simulink library "Linkage_DW_A"  (R2026a)
settings: Solver=VariableStepAuto
undefined symbols (not defined in the file): Ac, Af, Ar, InitLinkage, Left, Linkage, Visual, X, Y, Z
libraries: sm_lib x49, Suspension_Utilities x22, Linkage_Shock x1, fl_lib x1, nesl_utility x1
(part 1 of 2)
Description:
  | Component of Simscape Vehicle Templates Library
  | 
  | Copyright 2018-2024 The MathWorks, Inc.
settings Model: Creator=smiller  LastModifiedBy=andrei

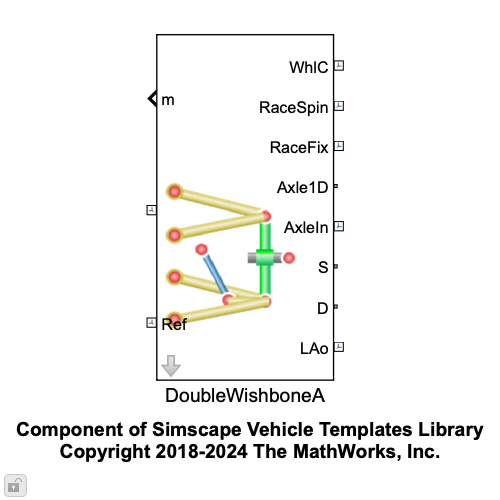
[thumbnail: Simulink's stored preview of the top-level diagram]
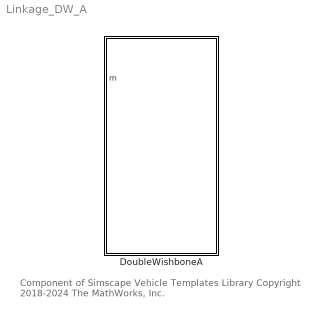
== system Linkage_DW_A ==
  note: Component of Simscape Vehicle Templates Library
      | Copyright 2018-2024 The MathWorks, Inc.
  DoubleWishboneA : Subsystem  VariantControl=DoubleWishboneA  mask(Double-Wishbone Suspension, Design A){popup_leftRight=Left, hp_in_f_ua=Linkage.UpperWishbone.sInboardF.Value, hp_in_r_ua=Linkage.UpperWishbone.sInboardR.Value, hp_out_ua=Linkage.UpperWishbone.sOutboard.Value, hp_in_f_la=Linkage.LowerWishbone.sInboardF.Value, hp_in_r_la=Linkage.LowerWishbone.sInboardR.Value, hp_out_la=Linkage.LowerWishbone.sOutboard.Value, hp_upr_cg=Linkage.Upright.sCG.Value, hp_upr_wc=Linkage.Upright.sWheelCentre.Value, hp_in_rod=Linkage.TrackRod.sInboard.Value, hp_upr_rod=Linkage.TrackRod.sOutboard.Value, hp_spr_top=Linkage.Shock.sTop.Value, hp_spr_bot=Linkage.Shock.sBottom.Value, clr_hp=Visual.hp.clr, opc_hp=Visual.hp.opc, size_hp=Visual.hp.rad, Upper_Arm_to_Subframe=Linkage.Upper_Arm_to_Subframe, ua_mass=Linkage.UpperWishbone.m.Value, clr_ua=Visual.UpperArm.clr, opc_ua=Visual.part.opc, radius_ua=Visual.UpperArm.rad, Lower_Arm_to_Subframe=Linkage.Lower_Arm_to_Subframe, la_mass=Linkage.LowerWishbone.m.Value, clr_la=Visual.LowerArm.clr, opc_la=Visual.part.opc, radius_la=Visual.LowerArm.rad, shock_pist_mass=Linkage.Shock.mPiston.Value, shock_cyl_mass=Linkage.Shock.mCylinder.Value, up_lim_bumpstop=Linkage.Endstop.xMax.Value, low_lim_bumpstop=Linkage.Endstop.xMin.Value, clr_conn_shock=Visual.hp.clr, opc_conn_shock=Visual.hp.opc, size_conn_shock=Visual.hp.rad, clr_shock_cyl=Visual.Shock.cyl.clr, opc_shock_cyl=Visual.part.opc, radius_shock_cyl=Visual.Shock.cyl.rad, clr_shock_piston=Visual.Shock.piston.clr, opc_shock_piston=Visual.part.opc, clr_shock_bumpstop=Visual.Shock.bumpstop.clr, opc_shock_bumpstop=Visual.part.opc, deadvol_len_shock_cyl=Visual.Shock.dead_length, piston_len_shock=Visual.Shock.piston.len, cyl_cap_len_shock=Visual.Shock.cap.len, bumpstop_len_shock=Visual.Shock.bumpstop.len, atoe=Linkage.Upright.aToe.Value, acamber=Linkage.Upright.aCamber.Value, upr_mass=Linkage.Upright.m.Value, axle_len=Linkage.Upright.xAxle.Value, axle_whlc_to_bearing=Linkage.Upright.xWCtoBearing.Value, axle_mass=Linkage.Upright.mAxle.Value, clr_conn_upr=Visual.hp.clr, opc_conn_upr=Visual.hp.opc, size_conn_upr=Visual.hp.rad, clr_upr=Visual.Upright.clr, opc_upr=Visual.part.opc, radius_upr=Visual.Upright.rad, clr_axle=Visual.Axle.clr, opc_axle=Visual.part.opc, radius_axle=Visual.Axle.rad, steer_class=Linkage.Steer.class.Value, rod_mass=Linkage.TrackRod.m.Value, clr_conn_rod=Visual.hp.clr, opc_conn_rod=Visual.hp.opc, size_conn_rod=Visual.hp.rad, clr_rod_str=Visual.SteeringArm.clr, opc_rod_str=Visual.part.opc, radius_rod_str=Visual.SteeringArm.rad, clr_rod=Visual.TrackRod.clr, opc_rod=Visual.part.opc, radius_rod=Visual.TrackRod.rad, whl_init_spd_lr=InitLinkage.nWheel.Value}
      mask prompts: popup_leftRight "Left/Right"; hp_in_f_ua "Upper Arm Front [xyz] (m)"; hp_in_r_ua "Upper Arm Rear [xyz] (m)"; hp_out_ua "Upper Arm Outboard [xyz] (m)"; hp_in_f_la "Lower Arm Front [xyz] (m)"; hp_in_r_la "Lower Arm Rear [xyz] (m)"; hp_out_la "Lower Arm Outboard [xyz] (m)"; hp_upr_cg "Upright CG [xyz] (m)"; hp_upr_wc "Wheel Center [xyz] (m)"; hp_in_rod "Track Rod Inboard [xyz] (m)"; hp_upr_rod "Track Rod Outboard [xyz] (m)"; hp_spr_top "Spring Top [xyz] (m)"; hp_spr_bot "Spring Bottom [xyz] (m)"; Upper_Arm_to_Subframe "Subframe Connection"; ua_mass "Mass (kg)"; clr_ua "Color [RGB]"; opc_ua "Opacity (0-1)"; radius_ua "Radius (m)"; Lower_Arm_to_Subframe "Subframe Connection"; la_mass "Mass (kg)"; clr_la "Color [RGB]"; opc_la "Opacity (0-1)"; radius_la "Radius (m)"; shock_pist_mass "Piston Mass (kg)"; shock_cyl_mass "Cylinder Mass (kg)"; up_lim_bumpstop "Upper Limit (m)"; low_lim_bumpstop "Lower Limit (m)"; deadvol_len_shock_cyl "Dead Volume Height (m)"; piston_len_shock "Piston Length (m)"; cyl_cap_len_shock "Cylinder Cap Length (m)"; bumpstop_len_shock "Bumpstop Length (m)"; atoe "Toe Angle (deg)"; acamber "Camber Angle (deg)"; upr_mass "Mass (kg)"; axle_len "Axle Length (m)"; axle_whlc_to_bearing "Distance Wheel Ctr to Bearing (m)"; axle_mass "Axle Mass (kg)"; steer_class "Steer (On/Off)"; rod_mass "Mass (kg)"; whl_init_spd_lr "Initial Wheel Speed (rad/s)"
      mask help: This models a double-wishbone suspension for steered and non-steered configurations. The non-steered configuration maintains its orientation via constraints attached to the upright.
      mask init:
      | curblk = gcb;
      | 
      | if(popup_leftRight == 1)
      |     rhs_susp = 1;
      |     %whlind = 1;
      |     whl_init_spd = whl_init_spd_lr(1);
      | elseif(popup_leftRight == 2)
      |     rhs_susp = -1;
      |     %whlind = 2;
      |     whl_init_spd = whl_init_spd_lr(2);
      | end
      | 
      | if(strcmpi(steer_class,'on'))
      |     %disp([curblk ': Turning Steering On'])
      |     set_param([curblk '/Track Rod'],'LabelModeActiveChoice','Steer')
      |     set_param([curblk '/LA Upright'],'LabelModeActiveChoice','Steer')
      |     set_param([gcb '/Rack'],'ForeGroundColor','black');
      | elseif(strcmpi(steer_class,'off'))
      |     %disp([curblk ': Turning Steering Off'])
      |     set_param([curblk '/Track Rod'],'LabelModeActiveChoice','No_Steer')
      |     set_param([curblk '/LA Upright'],'LabelModeActiveChoice','No_Steer')
      |     set_param([gcb '/Rack'],'ForeGroundColor','white');
      | end
      | 
      | %{
      | if(popup_conn_la == 1)
      |     set_param([gcb '/HP LA'],'LabelModeActiveChoice','Rigid_1Rev');
      | elseif(popup_conn_la == 2)
      |     set_param([gcb '/HP LA'],'LabelModeActiveChoice','Rigid_2Rev');
      | elseif(popup_conn_la == 3)
      |     set_param([gcb '/HP LA'],'LabelModeActiveChoice','Bushings');
      | end
      | 
      | if(popup_conn_ua == 1)
      |     set_param([gcb '/HP UA'],'LabelModeActiveChoice','Rigid_1Rev');
      | elseif(popup_conn_ua == 2)
      |     set_param([gcb '/HP UA'],'LabelModeActiveChoice','Rigid_2Rev');
      | elseif(popup_conn_ua == 3)
      |     set_param([gcb '/HP UA'],'LabelModeActiveChoice','Bushings');
      | end
      | %}
      mask Help: web('sm_car_double_wishbone_suspension_help.html')
      mask TypeOptions popup_leftRight: Hardpoints/popup_leftRight | Lower Arm/popup_leftRight | Upper Arm/popup_leftRight | Upright/popup_leftRight | Track Rod/Track Rod/popup_leftRight
      mask TypeOptions hp_in_f_ua: Upper Arm/hp_in_f | Hardpoints/hp_in_f_ua
      mask TypeOptions hp_in_r_ua: Upper Arm/hp_in_r | Hardpoints/hp_in_r_ua
      mask TypeOptions hp_out_ua: Upper Arm/hp_out | Upright/hp_ua_out
      mask TypeOptions hp_in_f_la: Lower Arm/hp_in_f | Hardpoints/hp_in_f_la
      mask TypeOptions hp_in_r_la: Lower Arm/hp_in_r | Hardpoints/hp_in_r_la
      mask TypeOptions hp_out_la: Lower Arm/hp_out | Upright/hp_la_out
      mask TypeOptions hp_upr_cg: Upright/hp_upr_cg
      mask TypeOptions hp_upr_wc: Upright/hp_upr_wc
      mask TypeOptions hp_in_rod: Track Rod/Track Rod/hp_in
      mask TypeOptions hp_upr_rod: Upright/hp_upr_rod | Track Rod/Track Rod/hp_out
      mask TypeOptions hp_spr_top: Hardpoints/hp_spr_top | Shock Absorber/hp_spr_top
      mask TypeOptions hp_spr_bot: Lower Arm/hp_spr | Shock Absorber/hp_spr_bot
      mask TypeOptions clr_hp: Hardpoints/clr_hp
      mask TypeOptions opc_hp: Hardpoints/opc_hp
      mask TypeOptions size_hp: Hardpoints/size_hp
      mask TypeOptions ua_mass: Upper Arm/ua_mass
      mask TypeOptions clr_ua: Upper Arm/clr_ua
      mask TypeOptions opc_ua: Upper Arm/opc_ua
      mask TypeOptions radius_ua: Upper Arm/radius_ua
      mask TypeOptions la_mass: Lower Arm/la_mass
      mask TypeOptions clr_la: Lower Arm/clr_la
      mask TypeOptions opc_la: Lower Arm/opc_la
      mask TypeOptions radius_la: Lower Arm/radius_la
      mask TypeOptions shock_pist_mass: Shock/shock_pist_mass
      mask TypeOptions shock_cyl_mass: Shock/shock_cyl_mass
      mask TypeOptions up_lim_bumpstop: Shock/up_lim_bumpstop
      mask TypeOptions low_lim_bumpstop: Shock/low_lim_bumpstop
      mask TypeOptions clr_conn_shock: Shock/clr_conn_shock
      mask TypeOptions opc_conn_shock: Shock/opc_conn_shock
      mask TypeOptions size_conn_shock: Shock/size_conn_shock
      mask TypeOptions clr_shock_cyl: Shock/clr_shock_cyl
      mask TypeOptions opc_shock_cyl: Shock/opc_shock_cyl
      mask TypeOptions radius_shock_cyl: Shock/radius_shock_cyl
      mask TypeOptions clr_shock_piston: Shock/clr_shock_piston
      mask TypeOptions opc_shock_piston: Shock/opc_shock_piston
      mask TypeOptions clr_shock_bumpstop: Shock/clr_shock_bumpstop
      mask TypeOptions opc_shock_bumpstop: Shock/opc_shock_bumpstop
      mask TypeOptions deadvol_len_shock_cyl: Shock/deadvol_len_shock_cyl
      mask TypeOptions piston_len_shock: Shock/piston_len_shock
      mask TypeOptions cyl_cap_len_shock: Shock/cyl_cap_len_shock
      mask TypeOptions bumpstop_len_shock: Shock/bumpstop_len_shock
      mask TypeOptions atoe: Upright/atoe
      mask TypeOptions acamber: Upright/acamber
      mask TypeOptions upr_mass: Upright/upr_mass
      mask TypeOptions axle_len: Upright/axle_len
      mask TypeOptions axle_whlc_to_bearing: Upright/axle_whlc_to_bearing
      mask TypeOptions axle_mass: Upright/axle_mass
      mask TypeOptions clr_conn_upr: Upright/clr_conn_upr
      mask TypeOptions opc_conn_upr: Upright/opc_conn_upr
      mask TypeOptions size_conn_upr: Upright/size_conn_upr
      mask TypeOptions clr_upr: Upright/clr_upr
      mask TypeOptions opc_upr: Upright/opc_upr
      mask TypeOptions radius_upr: Upright/radius_upr
      mask TypeOptions clr_axle: Upright/clr_axle
      mask TypeOptions opc_axle: Upright/opc_axle
      mask TypeOptions radius_axle: Upright/radius_axle
      mask TypeOptions rod_mass: Track Rod/Track Rod/rod_mass
      mask TypeOptions clr_conn_rod: Track Rod/Track Rod/clr_conn_rod
      mask TypeOptions opc_conn_rod: Track Rod/Track Rod/opc_conn_rod
      mask TypeOptions size_conn_rod: Track Rod/Track Rod/size_conn_rod
      mask TypeOptions clr_rod_str: Track Rod/Track Rod/clr_rod_str
      mask TypeOptions opc_rod_str: Track Rod/Track Rod/opc_rod_str
      mask TypeOptions radius_rod_str: Steer/CylinderRadius | Track Rod/Track Rod/radius_rod_str
      mask TypeOptions clr_rod: Track Rod/Track Rod/clr_rod
      mask TypeOptions opc_rod: Track Rod/Track Rod/opc_rod
      mask TypeOptions radius_rod: Track Rod/Track Rod/radius_rod
      mask DialogControl cont_hp Prompt: Hardpoints
      mask DialogControl cont_vis_hp Prompt: Visualization
      mask DialogControl text_clr_hp Prompt: Color [RGB]
      mask DialogControl text_opc_hp Prompt: Opac. (0-1)
      mask DialogControl text_size_hp Prompt: Size (m)
      mask DialogControl text_hp Prompt: Hardpoints
      mask DialogControl cont_ua Prompt: UA
      mask DialogControl cont_vis_ua Prompt: Visualization
      mask DialogControl cont_la Prompt: LA
      mask DialogControl cont_vis_la Prompt: Visualization
      mask DialogControl cont_shock Prompt: Shock
      mask DialogControl cont_parts Prompt: Parts
      mask DialogControl cont_bumpstop Prompt: Bumpstop
      mask DialogControl cont_vis_shock Prompt: Visualization
      mask DialogControl text_clr_shock Prompt: Color  [RGB]
      mask DialogControl text_opc_shock Prompt: Opac. (0-1)
      mask DialogControl text_size_shock Prompt: Size (m)
      mask DialogControl text_conn_shock Prompt: Connections
      mask DialogControl text_shock_shock Prompt: Cylinder
      mask DialogControl text_shock_piston Prompt: Piston
      mask DialogControl text_piston_radius Prompt: <cylinder radius>
      mask DialogControl text_shock_bumpstop Prompt: Bumpstop
      mask DialogControl text_bumpstop_radius Prompt: <cylinder radius>
      mask DialogControl cont_upright Prompt: Upright
      mask DialogControl grp_upright Prompt: Upright
      mask DialogControl grp_upright_axle Prompt: Axle
      mask DialogControl cont_vis_upr Prompt: Visualization
      mask DialogControl text_clr_upr Prompt: Color [RGB]
      mask DialogControl text_opc_upr Prompt: Opac. (0-1)
      mask DialogControl text_size_upr Prompt: Size (m)
      mask DialogControl text_conn_upr Prompt: Connections
      mask DialogControl text_upright Prompt: Upright
      mask DialogControl text_axle Prompt: Axle
      mask DialogControl cont_steer Prompt: Steer
      mask DialogControl grp_rod Prompt: Rod
      mask DialogControl cont_vis_rod Prompt: Visualization
      mask DialogControl text_clr_rod Prompt: Color [RGB]
      mask DialogControl text_opc_rod Prompt: Opac. (0-1)
      mask DialogControl text_size_rod Prompt: Size (m)
      mask DialogControl text_conn_rod Prompt: Connections
      mask DialogControl text_strarm Prompt: Steering Arm
      mask DialogControl text_rod_rod Prompt: Rod
      mask DialogControl cont_initial Prompt: Initial
      mask Display: image('sm_car_vehicle_linkage_dwa_IMAGE.png');

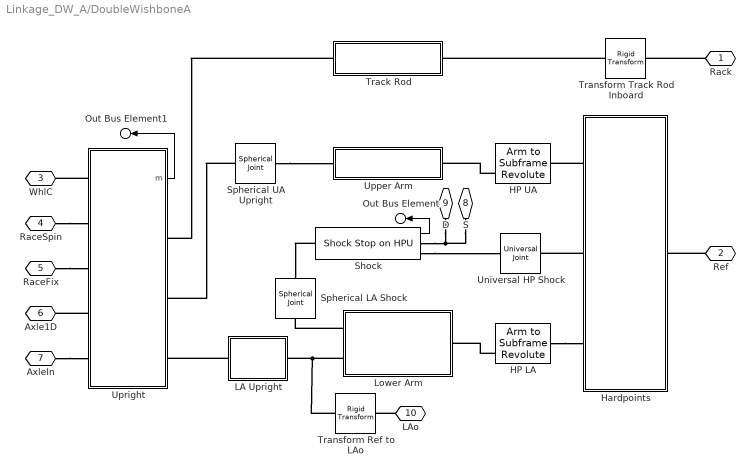
== system Linkage_DW_A/DoubleWishboneA ==
  HP LA : Suspension_Utilities/Arm to Subframe Revolute  VariantControl=Variant1  LabelModeActiveChoice=Rigid_1Rev  popup_leftRight=Left  hp_f=hp_in_f_ua  hp_r=hp_in_r_ua  Connection=Lower_Arm_to_Subframe  VariantLabel=Lower_Arm_to_Subframe.class.Value
      settings: AttributesFormatString=%<ActiveVariant>  SourceProductName=SmCar - Suspension Utilites
  HP UA : Suspension_Utilities/Arm to Subframe Revolute  VariantControl=Variant1  LabelModeActiveChoice=Rigid_1Rev  popup_leftRight=Left  hp_f=hp_in_f_ua  hp_r=hp_in_r_ua  Connection=Upper_Arm_to_Subframe  VariantLabel=Upper_Arm_to_Subframe.class.Value
      settings: AttributesFormatString=%<ActiveVariant>  SourceProductName=SmCar - Suspension Utilites
  Hardpoints : Subsystem  mask{popup_leftRight=Left, hp_in_f_ua=hp_in_f_ua, hp_in_r_ua=hp_in_r_ua, hp_in_f_la=hp_in_f_la, hp_in_r_la=hp_in_r_la, hp_spr_top=hp_spr_top, clr_hp=clr_hp, opc_hp=opc_hp, size_hp=size_hp}
      mask prompts: popup_leftRight "Left/Right"; hp_in_f_ua "Upper Arm Front [xyz] (m)"; hp_in_r_ua "Upper Arm Rear [xyz] (m)"; hp_in_f_la "Lower Arm Front [xyz] (m)"; hp_in_r_la "Lower Arm Rear [xyz] (m)"; hp_spr_top "Spring [xyz] (m)"
      mask init:
      | % Set parameter for mirroring (+y or -y)
      | if(popup_leftRight == 1)
      |     rhs_susp = 1;    
      | elseif(popup_leftRight == 2)
      |     rhs_susp = -1;
      | end
      | 
      | rhs_hp = [1 rhs_susp 1];
      mask TypeOptions popup_leftRight: Left | Right
      mask TypeOptions clr_hp: Subsystem/Vis HP LAf/GraphicDiffuseColor | Vis HP LAr/GraphicDiffuseColor | Vis HP Spring/GraphicDiffuseColor | Vis HP UAf/GraphicDiffuseColor | Vis HP UAr/GraphicDiffuseColor
      mask TypeOptions opc_hp: Subsystem/Vis HP LAf/GraphicOpacity | Vis HP LAr/GraphicOpacity | Vis HP Spring/GraphicOpacity | Vis HP UAf/GraphicOpacity | Vis HP UAr/GraphicOpacity
      mask DialogControl cont_hp Prompt: Hardpoints
      mask DialogControl cont_vis_hp Prompt: Visualization
      mask DialogControl text_clr_hp Prompt: Color [RGB]
      mask DialogControl text_opc_hp Prompt: Opac. (0-1)
      mask DialogControl text_size_hp Prompt: Size (m)
      mask DialogControl text_hp Prompt: Hardpoints
      mask Display: image('sm_car_vehicle_linkage_dw_hp_IMAGE.png');
  LA Upright : Subsystem  Variant=on  VariantControlMode=label  VariantControl=Variant1  LabelModeActiveChoice=No_Steer
      settings: AttributesFormatString=%<ActiveVariant>
  Lower Arm : Subsystem  mask(Lower Arm (Wishbone)){popup_leftRight=Left, hp_in_f=hp_in_f_la, hp_in_r=hp_in_r_la, hp_out=hp_out_la, hp_spr=hp_spr_bot, la_mass=la_mass, clr_la=clr_la, opc_la=opc_la, radius_la=radius_la}
      mask prompts: popup_leftRight "Left/Right"; hp_in_f "Inboard Front [xyz] (m)"; hp_in_r "Inboard Rear [xyz] (m)"; hp_out "Outboard [xyz] (m)"; hp_spr "Spring [xyz] (m)"; la_mass "Mass (kg)"; clr_la "Color [RGB]"; opc_la "Opacity (0-1)"; radius_la "Radius (m)"
      mask help: This subsystem models the lower arm of a wishbone suspension. It can be configured to have one or two attachment points to the chassis. There are connections to the upright and spring.
      mask init:
      | % Set parameter for mirroring (+y or -y)
      | if(popup_leftRight == 1)
      |     rhs_susp = 1;
      | elseif(popup_leftRight == 2)
      |     rhs_susp = -1;
      | end
      | 
      | rhs_hp = [1 rhs_susp 1];
      mask Help: web ('sm_car_lower_arm_help.html')
      mask TypeOptions popup_leftRight: Left | Right
      mask TypeOptions clr_la: Arm F/clr_solid | Arm R/clr_solid | Arm Spring/clr_solid
      mask TypeOptions opc_la: Arm F/opc_solid | Arm R/opc_solid | Arm Spring/opc_solid
      mask TypeOptions radius_la: Arm F/rad_solid | Arm R/rad_solid | Arm Spring/rad_solid
      mask DialogControl cont_ua Prompt: LA
      mask DialogControl cont_vis_la Prompt: Visualization
      mask Display: image('sm_car_vehicle_linkage_dw_la_IMAGE.png');
  Shock : Linkage_Shock/Shock Stop on HPU  shock_pist_mass=shock_pist_mass  shock_cyl_mass=shock_cyl_mass  hp_spr_top=hp_spr_top  hp_spr_bot=hp_spr_bot  up_lim_bumpstop=up_lim_bumpstop  low_lim_bumpstop=low_lim_bumpstop  clr_conn_shock=clr_conn_shock  opc_conn_shock=opc_conn_shock  size_conn_shock=size_conn_shock  clr_shock_cyl=clr_shock_cyl  opc_shock_cyl=opc_shock_cyl  radius_shock_cyl=radius_shock_cyl  clr_shock_piston=clr_shock_piston  opc_shock_piston=opc_shock_piston  clr_shock_bumpstop=clr_shock_bumpstop  opc_shock_bumpstop=opc_shock_bumpstop  deadvol_len_shock_cyl=deadvol_len_shock_cyl  piston_len_shock=piston_len_shock  cyl_cap_len_shock=cyl_cap_len_shock  bumpstop_len_shock=bumpstop_len_shock
  Spherical LA Shock : sm_lib/Joints/Spherical Joint  JointMode=Normal  CompositeWrenchDir=FollowerOnBase  CompositeWrenchFrame=BaseFrame  SenseConstraintForce=off  SenseConstraintTorque=off  SenseTotalForce=off  SenseTotalTorque=off  PositionTargetSpecify=off  PositionTargetPriority=High  PositionTargetRotationMethod=None  PositionTargetFollAlignAxisA=+X  PositionTargetBaseAlignAxisA=+Y  PositionTargetFollAlignAxisB=+Y  PositionTargetBaseAlignAxisB=+Z  PositionTargetRotationStandardAxis=+Z  PositionTargetRotationAngle=0.0  PositionTargetRotationAngleUnits=deg  PositionTargetRotationArbitraryAxis=[0 0 1]  PositionTargetRotationSequenceAxes=FollowerAxes  PositionTargetRotationSequence=XYX  PositionTargetRotationSequenceAngles=[0 0 0]  PositionTargetRotationSequenceAnglesUnits=deg  PositionTargetRotationMatrix=[1 0 0; 0 1 0; 0 0 1]  PositionTargetQuaternion=[1 0 0 0]  VelocityTargetSpecify=off  VelocityTargetPriority=High  VelocityTargetValue=[0 0 0]  VelocityTargetValueUnits=deg/s  VelocityTargetInFollowerFrame=on  EqPosRotationMethod=None  EqPosFollAlignAxisA=+X  EqPosBaseAlignAxisA=+Y  EqPosFollAlignAxisB=+Y  EqPosBaseAlignAxisB=+Z  EqPosRotationStandardAxis=+Z  EqPosRotationAngle=0.0  EqPosRotationAngleUnits=deg  EqPosRotationArbitraryAxis=[0 0 1]  EqPosRotationSequenceAxes=FollowerAxes  EqPosRotationSequence=XYX  EqPosRotationSequenceAngles=[0 0 0]  EqPosRotationSequenceAnglesUnits=deg  EqPosRotationMatrix=[1 0 0; 0 1 0; 0 0 1]  EqPosQuaternion=[1 0 0 0]  SpringStiffness=0  SpringStiffnessUnits=N*m/deg  DampingCoefficient=0  DampingCoefficientUnits=N*m/(deg/s)  LowerLimitSpecify=off  LowerLimitBound=15  LowerLimitBoundUnits=deg  LowerLimitStiffness=1e4  LowerLimitStiffnessUnits=N*m/deg  LowerLimitDamping=10  LowerLimitDampingUnits=N*m/(deg/s)  LowerLimitTransitionRegionWidth=0.1  LowerLimitTransitionRegionWidthUnits=deg  UpperLimitSpecify=off  UpperLimitBound=45  UpperLimitBoundUnits=deg  UpperLimitStiffness=1e4  UpperLimitStiffnessUnits=N*m/deg  UpperLimitDamping=10  UpperLimitDampingUnits=N*m/(deg/s)  UpperLimitTransitionRegionWidth=0.1  UpperLimitTransitionRegionWidthUnits=deg  TorqueActuationMode=NoTorque  ActuateTorqueX=off  ActuateTorqueY=off  ActuateTorqueZ=off  ActuateTorque=off  ActuationFrame=BaseFrame  SensePosition=off  SenseVelocityX=off  SenseVelocityY=off  SenseVelocityZ=off  SenseVelocity=off  SenseAccelerationX=off  SenseAccelerationY=off  SenseAccelerationZ=off  SenseAcceleration=off  SenseLowerLimitTorqueMag=off  SenseUpperLimitTorqueMag=off  SensingFrame=BaseFrame
  Spherical UA Upright : sm_lib/Joints/Spherical Joint  JointMode=Normal  CompositeWrenchDir=FollowerOnBase  CompositeWrenchFrame=BaseFrame  SenseConstraintForce=off  SenseConstraintTorque=off  SenseTotalForce=off  SenseTotalTorque=off  PositionTargetSpecify=on  PositionTargetPriority=High  PositionTargetRotationMethod=StandardAxis  PositionTargetFollAlignAxisA=+X  PositionTargetBaseAlignAxisA=+Y  PositionTargetFollAlignAxisB=+Y  PositionTargetBaseAlignAxisB=+Z  PositionTargetRotationStandardAxis=+Z  PositionTargetRotationAngle=0.0  PositionTargetRotationAngleUnits=deg  PositionTargetRotationArbitraryAxis=[0 0 1]  PositionTargetRotationSequenceAxes=FollowerAxes  PositionTargetRotationSequence=XYX  PositionTargetRotationSequenceAngles=[0 0 0]  PositionTargetRotationSequenceAnglesUnits=deg  PositionTargetRotationMatrix=[1 0 0; 0 1 0; 0 0 1]  PositionTargetQuaternion=[1 0 0 0]  VelocityTargetSpecify=off  VelocityTargetPriority=High  VelocityTargetValue=[0 0 0]  VelocityTargetValueUnits=deg/s  VelocityTargetInFollowerFrame=on  EqPosRotationMethod=None  EqPosFollAlignAxisA=+X  EqPosBaseAlignAxisA=+Y  EqPosFollAlignAxisB=+Y  EqPosBaseAlignAxisB=+Z  EqPosRotationStandardAxis=+Z  EqPosRotationAngle=0.0  EqPosRotationAngleUnits=deg  EqPosRotationArbitraryAxis=[0 0 1]  EqPosRotationSequenceAxes=FollowerAxes  EqPosRotationSequence=XYX  EqPosRotationSequenceAngles=[0 0 0]  EqPosRotationSequenceAnglesUnits=deg  EqPosRotationMatrix=[1 0 0; 0 1 0; 0 0 1]  EqPosQuaternion=[1 0 0 0]  SpringStiffness=0  SpringStiffnessUnits=N*m/deg  DampingCoefficient=0  DampingCoefficientUnits=N*m/(deg/s)  LowerLimitSpecify=off  LowerLimitBound=15  LowerLimitBoundUnits=deg  LowerLimitStiffness=1e4  LowerLimitStiffnessUnits=N*m/deg  LowerLimitDamping=10  LowerLimitDampingUnits=N*m/(deg/s)  LowerLimitTransitionRegionWidth=0.1  LowerLimitTransitionRegionWidthUnits=deg  UpperLimitSpecify=off  UpperLimitBound=45  UpperLimitBoundUnits=deg  UpperLimitStiffness=1e4  UpperLimitStiffnessUnits=N*m/deg  UpperLimitDamping=10  UpperLimitDampingUnits=N*m/(deg/s)  UpperLimitTransitionRegionWidth=0.1  UpperLimitTransitionRegionWidthUnits=deg  TorqueActuationMode=NoTorque  ActuateTorqueX=off  ActuateTorqueY=off  ActuateTorqueZ=off  ActuateTorque=off  ActuationFrame=BaseFrame  SensePosition=off  SenseVelocityX=off  SenseVelocityY=off  SenseVelocityZ=off  SenseVelocity=off  SenseAccelerationX=off  SenseAccelerationY=off  SenseAccelerationZ=off  SenseAcceleration=off  SenseLowerLimitTorqueMag=off  SenseUpperLimitTorqueMag=off  SensingFrame=BaseFrame
  Track Rod : Subsystem  Variant=on  VariantControlMode=label  VariantControl=Variant1  LabelModeActiveChoice=No_Steer
      settings: AttributesFormatString=%<ActiveVariant>
  Transform Ref to LAo : sm_lib/Frames and Transforms/Rigid Transform  RotationMethod=None  FollAlignAxisA=+X  BaseAlignAxisA=+Y  FollAlignAxisB=+Y  BaseAlignAxisB=+Z  RotationStandardAxis=+Z  RotationAngle=0.0  RotationAngleUnits=deg  RotationArbitraryAxis=[0 0 1]  RotationSequenceAxes=FollowerAxes  RotationSequence=XYX  RotationSequenceAngles=[0 0 0]  RotationSequenceAnglesUnits=deg  RotationMatrix=[1 0 0; 0 1 0; 0 0 1]  Quaternion=[1 0 0 0]  TranslationMethod=Cartesian  TranslationCartesianOffset=hp_out_la.*[1 rhs_susp 1]  TranslationCartesianOffsetUnits=m  TranslationStandardAxis=+Z  TranslationStandardOffset=0  TranslationStandardOffsetUnits=m  TranslationROffset=0  TranslationROffsetUnits=m  TranslationThetaOffset=0  TranslationThetaOffsetUnits=deg  TranslationZOffset=0  TranslationZOffsetUnits=m
  Transform Track Rod Inboard : sm_lib/Frames and Transforms/Rigid Transform  RotationMethod=None  FollAlignAxisA=+X  BaseAlignAxisA=+Y  FollAlignAxisB=+Y  BaseAlignAxisB=+Z  RotationStandardAxis=+Z  RotationAngle=0.0  RotationAngleUnits=deg  RotationArbitraryAxis=[0 0 1]  RotationSequenceAxes=FollowerAxes  RotationSequence=XYX  RotationSequenceAngles=[0 0 0]  RotationSequenceAnglesUnits=deg  RotationMatrix=[1 0 0; 0 1 0; 0 0 1]  Quaternion=[1 0 0 0]  TranslationMethod=Cartesian  TranslationCartesianOffset=hp_in_rod.*[1 rhs_susp 1]  TranslationCartesianOffsetUnits=m  TranslationStandardAxis=+Z  TranslationStandardOffset=0  TranslationStandardOffsetUnits=m  TranslationROffset=0  TranslationROffsetUnits=m  TranslationThetaOffset=0  TranslationThetaOffsetUnits=deg  TranslationZOffset=0  TranslationZOffsetUnits=m
  Universal HP Shock : sm_lib/Joints/Universal Joint  JointMode=Normal  CompositeWrenchDir=FollowerOnBase  CompositeWrenchFrame=BaseFrame  SenseConstraintForce=off  SenseConstraintTorque=off  SenseTotalForce=off  SenseTotalTorque=off  RxPositionTargetSpecify=off  RxPositionTargetPriority=High  RxPositionTargetValue=0  RxPositionTargetValueUnits=deg  RxVelocityTargetSpecify=off  RxVelocityTargetPriority=High  RxVelocityTargetValue=0  RxVelocityTargetValueUnits=deg/s  RxEquilibriumPosition=0  RxEquilibriumPositionUnits=deg  RxSpringStiffness=0  RxSpringStiffnessUnits=N*m/deg  RxDampingCoefficient=0  RxDampingCoefficientUnits=N*m/(deg/s)  RxLowerLimitSpecify=off  RxLowerLimitBound=-90  RxLowerLimitBoundUnits=deg  RxLowerLimitStiffness=1e4  RxLowerLimitStiffnessUnits=N*m/deg  RxLowerLimitDamping=10  RxLowerLimitDampingUnits=N*m/(deg/s)  RxLowerLimitTransitionRegionWidth=0.1  RxLowerLimitTransitionRegionWidthUnits=deg  RxUpperLimitSpecify=off  RxUpperLimitBound=90  RxUpperLimitBoundUnits=deg  RxUpperLimitStiffness=1e4  RxUpperLimitStiffnessUnits=N*m/deg  RxUpperLimitDamping=10  RxUpperLimitDampingUnits=N*m/(deg/s)  RxUpperLimitTransitionRegionWidth=0.1  RxUpperLimitTransitionRegionWidthUnits=deg  RxTorqueActuationMode=NoTorque  RxMotionActuationMode=ComputedMotion  RxSensePosition=off  RxSenseVelocity=off  RxSenseAcceleration=off  RxSenseTorqueForce=off  RxSenseLowerLimitTorqueForce=off  RxSenseUpperLimitTorqueForce=off  RyPositionTargetSpecify=off  RyPositionTargetPriority=High  RyPositionTargetValue=0  RyPositionTargetValueUnits=deg  RyVelocityTargetSpecify=off  RyVelocityTargetPriority=High  RyVelocityTargetValue=0  RyVelocityTargetValueUnits=deg/s  RyEquilibriumPosition=0  RyEquilibriumPositionUnits=deg  RySpringStiffness=0  RySpringStiffnessUnits=N*m/deg  RyDampingCoefficient=0  RyDampingCoefficientUnits=N*m/(deg/s)  RyLowerLimitSpecify=off  RyLowerLimitBound=-90  RyLowerLimitBoundUnits=deg  RyLowerLimitStiffness=1e4  RyLowerLimitStiffnessUnits=N*m/deg  RyLowerLimitDamping=10  RyLowerLimitDampingUnits=N*m/(deg/s)  RyLowerLimitTransitionRegionWidth=0.1  RyLowerLimitTransitionRegionWidthUnits=deg  RyUpperLimitSpecify=off  RyUpperLimitBound=90  RyUpperLimitBoundUnits=deg  RyUpperLimitStiffness=1e4  RyUpperLimitStiffnessUnits=N*m/deg  RyUpperLimitDamping=10  RyUpperLimitDampingUnits=N*m/(deg/s)  RyUpperLimitTransitionRegionWidth=0.1  RyUpperLimitTransitionRegionWidthUnits=deg  RyTorqueActuationMode=NoTorque  RyMotionActuationMode=ComputedMotion  RySensePosition=off  RySenseVelocity=off  RySenseAcceleration=off  RySenseTorqueForce=off  RySenseLowerLimitTorqueForce=off  RySenseUpperLimitTorqueForce=off
  Upper Arm : Subsystem  mask{popup_leftRight=Left, hp_in_f=hp_in_f_ua, hp_in_r=hp_in_r_ua, hp_out=hp_out_ua, ua_mass=ua_mass, clr_ua=clr_ua, opc_ua=opc_ua, radius_ua=radius_ua}
      mask prompts: popup_leftRight "Left/Right"; hp_in_f "Inboard Front [xyz] (m)"; hp_in_r "Inboard Rear [xyz] (m)"; hp_out "Outboard [xyz] (m)"; ua_mass "Mass (kg)"; clr_ua "Color [RGB]"; opc_ua "Opacity (0-1)"; radius_ua "Radius (m)"
      mask init:
      | if(popup_leftRight == 1)
      |     rhs_susp = 1;
      | elseif(popup_leftRight == 2)
      |     rhs_susp = -1;
      | end
      | 
      | rhs_hp = [1 rhs_susp 1];
      mask TypeOptions popup_leftRight: Left | Right
      mask TypeOptions clr_ua: Arm F/clr_solid | Arm R/clr_solid
      mask TypeOptions opc_ua: Arm F/opc_solid | Arm R/opc_solid
      mask TypeOptions radius_ua: Arm F/rad_solid | Arm R/rad_solid
      mask DialogControl cont_ua Prompt: UA
      mask DialogControl cont_vis_ua Prompt: Visualization
      mask Display: image('sm_car_vehicle_linkage_dw_ua_IMAGE.png');
  Upright : Subsystem  mask{popup_leftRight=Left, hp_ua_out=hp_out_ua, hp_la_out=hp_out_la, hp_upr_rod=hp_upr_rod, hp_upr_cg=hp_upr_cg, hp_upr_wc=hp_upr_wc, axle_len=axle_len, axle_whlc_to_bearing=axle_whlc_to_bearing, axle_mass=axle_mass, atoe=atoe, acamber=acamber, upr_mass=upr_mass, whl_init_spd_upr=whl_init_spd, clr_conn_upr=clr_conn_upr, opc_conn_upr=opc_conn_upr, size_conn_upr=size_conn_upr, clr_upr=clr_upr, opc_upr=opc_upr, radius_upr=radius_upr, clr_axle=clr_axle, opc_axle=opc_axle, radius_axle=radius_axle}
      mask prompts: popup_leftRight "Left/Right"; hp_ua_out "Upper Arm Outboard [xyz] (m)"; hp_la_out "Lower Arm Outboard [xyz] (m)"; hp_upr_rod "Track Rod Outboard [xyz] (m)"; hp_upr_cg "Center of Mass [xyz] (m)"; hp_upr_wc "Wheel Center [xyz] (m)"; axle_len "Axle Length (m)"; axle_whlc_to_bearing "Distance Wheel Ctr to Bearing (m)"; axle_mass "Axle Mass (kg)"; atoe "Toe Angle (deg)"; acamber "Camber Angle (deg)"; upr_mass "Upright Mass (kg)"; whl_init_spd_upr "Initial Wheel Speed (rad/s)"
      mask init:
      | % Set parameter for mirroring (+y or -y)
      | if(popup_leftRight == 1)
      |     rhs_upr = 1;
      | elseif(popup_leftRight == 2)
      |     rhs_upr = -1;
      | end
      | rhs_hp = [1 rhs_upr 1];
      | 
      | % Additional hardpoint at center of upright
      | % Used as attachment points for axle and steering arm
      | hp_upr_ctr = (hp_ua_out+hp_la_out)/2;
      mask TypeOptions popup_leftRight: Left | Right
      mask TypeOptions axle_mass: Axle/Mass
      mask TypeOptions upr_mass:
      | Inertia
      | CG/Mass
      mask TypeOptions whl_init_spd_upr: Revolute/whl_init_spd_jnt
      mask TypeOptions clr_conn_upr:
      | Vis Upright LA/GraphicDiffuseColor | Vis Upright UA/GraphicDiffuseColor | Vis Wheel
      | Center/GraphicDiffuseColor
      mask TypeOptions opc_conn_upr:
      | Vis Upright LA/GraphicOpacity | Vis Upright UA/GraphicOpacity | Vis Wheel
      | Center/GraphicOpacity
      mask TypeOptions clr_upr: Upright/clr_solid | Steering Arm/clr_solid
      mask TypeOptions opc_upr: Upright/opc_solid | Steering Arm/opc_solid
      mask TypeOptions radius_upr: Upright/rad_solid | Steering Arm/rad_solid
      mask TypeOptions clr_axle: Axle/GraphicDiffuseColor
      mask TypeOptions opc_axle: Axle/GraphicOpacity
      mask TypeOptions radius_axle: Axle/CylinderRadius
      mask DialogControl cont_upright Prompt: Upright
      mask DialogControl grp_upright Prompt: Initialization
      mask DialogControl cont_vis_upr Prompt: Visualization
      mask DialogControl text_clr_upr Prompt: Color [RGB]
      mask DialogControl text_opc_upr Prompt: Opac. (0-1)
      mask DialogControl text_size_upr Prompt: Size (m)
      mask DialogControl text_conn_upr Prompt: Connections
      mask DialogControl text_upright Prompt: Upright
      mask DialogControl text_axle Prompt: Axle
      mask Display: image('sm_car_vehicle_linkage_dw_upr_IMAGE.png');
  Rack : PMIOPort  Side=Right
  Ref : PMIOPort  Port=2  Side=Right
  WhlC : PMIOPort  Port=3  Side=Left
  RaceSpin : PMIOPort  Port=4  Side=Left
  RaceFix : PMIOPort  Port=5  Side=Left
  Axle1D : PMIOPort  Port=6  Side=Left
  AxleIn : PMIOPort  Port=7  Side=Left
  S : PMIOPort  Port=8  Side=Left
  D : PMIOPort  Port=9  Side=Left
  LAo : PMIOPort  Port=10  Side=Left
  Out Bus Element : Outport  VectorParamsAs1DForOutWhenUnconnected=off  PortName=m  Element=Shock
  Out Bus Element1 : Outport  VectorParamsAs1DForOutWhenUnconnected=off  PortName=m  Element=Upright
  wires:
  Shock/1 -> Out Bus Element/1
  Upright/1(m) -> Out Bus Element1/1
  connections:
  AxleIn/RConn1 -- Upright/LConn5
  RaceFix/RConn1 -- Upright/LConn3
  RaceSpin/RConn1 -- Upright/LConn2
  Spherical UA Upright/RConn1 -- Upright/RConn2
  Lower Arm/LConn2 -- Transform Ref to LAo/RConn1 -- LA Upright/LConn1
  HP LA/RConn1 -- Lower Arm/RConn1
  Spherical UA Upright/LConn1 -- Upper Arm/LConn1
  LA Upright/RConn1 -- Upright/RConn3
  Lower Arm/LConn1 -- Spherical LA Shock/LConn1
  HP LA/LConn1 -- Hardpoints/LConn3
  HP UA/RConn1 -- Upper Arm/RConn1
  S/RConn1 -- D/RConn1 -- Shock/RConn1
  Upright/LConn4 -- Axle1D/RConn1
  Transform Track Rod Inboard/RConn1 -- Track Rod/RConn1
  Track Rod/LConn1 -- Upright/RConn1
  Hardpoints/LConn1 -- HP UA/LConn1
  Ref/RConn1 -- Hardpoints/RConn1
  Hardpoints/LConn2 -- Universal HP Shock/LConn1
  Shock/LConn1 -- Spherical LA Shock/RConn1
  Upright/LConn1 -- WhlC/RConn1
  Shock/RConn2 -- Universal HP Shock/RConn1
  Rack/RConn1 -- Transform Track Rod Inboard/LConn1
  LAo/RConn1 -- Transform Ref to LAo/LConn1

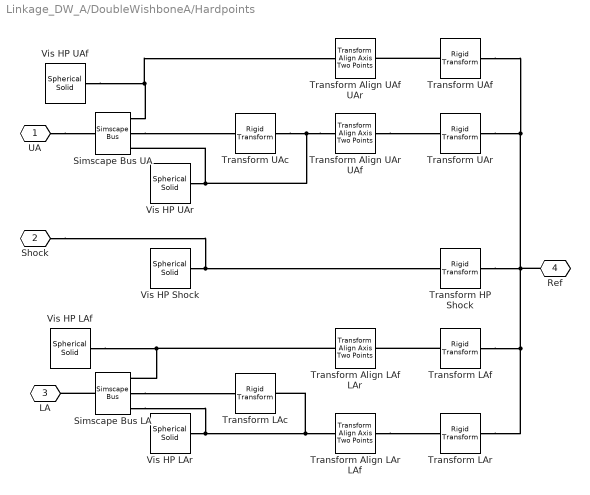
== system Linkage_DW_A/DoubleWishboneA/Hardpoints ==
  Simscape Bus LA : SimscapeBus  HierarchyStrings=Af;Ac;Ar
  Simscape Bus UA : SimscapeBus  HierarchyStrings=Af;Ac;Ar
  Transform Align LAf LAr : Suspension_Utilities/Transform Align Axis Two Points  hp_b=hp_in_f_la.*rhs_hp  hp_t=hp_in_r_la.*rhs_hp  popup_f_axis=-Z
      settings: SourceProductName=SmCar - Suspension Utilites
  Transform Align LAr LAf : Suspension_Utilities/Transform Align Axis Two Points  hp_b=hp_in_r_la.*rhs_hp  hp_t=hp_in_f_la.*rhs_hp  popup_f_axis=+Z
      settings: SourceProductName=SmCar - Suspension Utilites
  Transform Align UAf UAr : Suspension_Utilities/Transform Align Axis Two Points  hp_b=hp_in_f_ua.*rhs_hp  hp_t=hp_in_r_ua.*rhs_hp  popup_f_axis=-Z
      settings: SourceProductName=SmCar - Suspension Utilites
  Transform Align UAr UAf : Suspension_Utilities/Transform Align Axis Two Points  hp_b=hp_in_r_ua.*rhs_hp  hp_t=hp_in_f_ua.*rhs_hp  popup_f_axis=+Z
      settings: SourceProductName=SmCar - Suspension Utilites
  Transform HP Shock : sm_lib/Frames and Transforms/Rigid Transform  RotationMethod=None  FollAlignAxisA=+X  BaseAlignAxisA=+Y  FollAlignAxisB=+Y  BaseAlignAxisB=+Z  RotationStandardAxis=+Z  RotationAngle=0.0  RotationAngleUnits=deg  RotationArbitraryAxis=[0 0 1]  RotationSequenceAxes=FollowerAxes  RotationSequence=XYX  RotationSequenceAngles=[0 0 0]  RotationSequenceAnglesUnits=deg  RotationMatrix=[1 0 0; 0 1 0; 0 0 1]  Quaternion=[1 0 0 0]  TranslationMethod=Cartesian  TranslationCartesianOffset=hp_spr_top.*rhs_hp  TranslationCartesianOffsetUnits=m  TranslationStandardAxis=+Z  TranslationStandardOffset=0  TranslationStandardOffsetUnits=m  TranslationROffset=0  TranslationROffsetUnits=m  TranslationThetaOffset=0  TranslationThetaOffsetUnits=deg  TranslationZOffset=0  TranslationZOffsetUnits=m
  Transform LAc : sm_lib/Frames and Transforms/Rigid Transform  RotationMethod=None  FollAlignAxisA=+X  BaseAlignAxisA=+Y  FollAlignAxisB=+Y  BaseAlignAxisB=+Z  RotationStandardAxis=+Z  RotationAngle=0  RotationAngleUnits=deg  RotationArbitraryAxis=[0 0 1]  RotationSequenceAxes=FollowerAxes  RotationSequence=XYX  RotationSequenceAngles=[0 0 0]  RotationSequenceAnglesUnits=deg  RotationMatrix=[0 0 -1;0 1 0;1 0 0]  Quaternion=[1 0 0 0]  TranslationMethod=StandardAxis  TranslationCartesianOffset=[0 0 0]  TranslationCartesianOffsetUnits=m  TranslationStandardAxis=+Z  TranslationStandardOffset=norm(hp_in_f_la-hp_in_r_la)/2  TranslationStandardOffsetUnits=m  TranslationROffset=0  TranslationROffsetUnits=m  TranslationThetaOffset=0  TranslationThetaOffsetUnits=deg  TranslationZOffset=0  TranslationZOffsetUnits=m
  Transform LAf : sm_lib/Frames and Transforms/Rigid Transform  RotationMethod=None  FollAlignAxisA=+X  BaseAlignAxisA=+Y  FollAlignAxisB=+Y  BaseAlignAxisB=+Z  RotationStandardAxis=+Z  RotationAngle=0.0  RotationAngleUnits=deg  RotationArbitraryAxis=[0 0 1]  RotationSequenceAxes=FollowerAxes  RotationSequence=XYX  RotationSequenceAngles=[0 0 0]  RotationSequenceAnglesUnits=deg  RotationMatrix=[1 0 0; 0 1 0; 0 0 1]  Quaternion=[1 0 0 0]  TranslationMethod=Cartesian  TranslationCartesianOffset=hp_in_f_la.*rhs_hp  TranslationCartesianOffsetUnits=m  TranslationStandardAxis=+Z  TranslationStandardOffset=0  TranslationStandardOffsetUnits=m  TranslationROffset=0  TranslationROffsetUnits=m  TranslationThetaOffset=0  TranslationThetaOffsetUnits=deg  TranslationZOffset=0  TranslationZOffsetUnits=m
  Transform LAr : sm_lib/Frames and Transforms/Rigid Transform  RotationMethod=None  FollAlignAxisA=+X  BaseAlignAxisA=+Y  FollAlignAxisB=+Y  BaseAlignAxisB=+Z  RotationStandardAxis=+Z  RotationAngle=0.0  RotationAngleUnits=deg  RotationArbitraryAxis=[0 0 1]  RotationSequenceAxes=FollowerAxes  RotationSequence=XYX  RotationSequenceAngles=[0 0 0]  RotationSequenceAnglesUnits=deg  RotationMatrix=[1 0 0; 0 1 0; 0 0 1]  Quaternion=[1 0 0 0]  TranslationMethod=Cartesian  TranslationCartesianOffset=hp_in_r_la.*rhs_hp  TranslationCartesianOffsetUnits=m  TranslationStandardAxis=+Z  TranslationStandardOffset=0  TranslationStandardOffsetUnits=m  TranslationROffset=0  TranslationROffsetUnits=m  TranslationThetaOffset=0  TranslationThetaOffsetUnits=deg  TranslationZOffset=0  TranslationZOffsetUnits=m
  Transform UAc : sm_lib/Frames and Transforms/Rigid Transform  RotationMethod=None  FollAlignAxisA=+X  BaseAlignAxisA=+Y  FollAlignAxisB=+Y  BaseAlignAxisB=+Z  RotationStandardAxis=+Z  RotationAngle=0  RotationAngleUnits=deg  RotationArbitraryAxis=[0 0 1]  RotationSequenceAxes=FollowerAxes  RotationSequence=XYX  RotationSequenceAngles=[0 0 0]  RotationSequenceAnglesUnits=deg  RotationMatrix=[0 0 -1;0 1 0;1 0 0]  Quaternion=[1 0 0 0]  TranslationMethod=StandardAxis  TranslationCartesianOffset=[0 0 0]  TranslationCartesianOffsetUnits=m  TranslationStandardAxis=+Z  TranslationStandardOffset=norm(hp_in_f_ua - hp_in_r_ua)/2  TranslationStandardOffsetUnits=m  TranslationROffset=0  TranslationROffsetUnits=m  TranslationThetaOffset=0  TranslationThetaOffsetUnits=deg  TranslationZOffset=0  TranslationZOffsetUnits=m
  Transform UAf : sm_lib/Frames and Transforms/Rigid Transform  RotationMethod=None  FollAlignAxisA=+X  BaseAlignAxisA=+Y  FollAlignAxisB=+Y  BaseAlignAxisB=+Z  RotationStandardAxis=+Z  RotationAngle=0.0  RotationAngleUnits=deg  RotationArbitraryAxis=[0 0 1]  RotationSequenceAxes=FollowerAxes  RotationSequence=XYX  RotationSequenceAngles=[0 0 0]  RotationSequenceAnglesUnits=deg  RotationMatrix=[1 0 0; 0 1 0; 0 0 1]  Quaternion=[1 0 0 0]  TranslationMethod=Cartesian  TranslationCartesianOffset=hp_in_f_ua.*rhs_hp  TranslationCartesianOffsetUnits=m  TranslationStandardAxis=+Z  TranslationStandardOffset=0  TranslationStandardOffsetUnits=m  TranslationROffset=0  TranslationROffsetUnits=m  TranslationThetaOffset=0  TranslationThetaOffsetUnits=deg  TranslationZOffset=0  TranslationZOffsetUnits=m
  Transform UAr : sm_lib/Frames and Transforms/Rigid Transform  RotationMethod=None  FollAlignAxisA=+X  BaseAlignAxisA=+Y  FollAlignAxisB=+Y  BaseAlignAxisB=+Z  RotationStandardAxis=+Z  RotationAngle=0.0  RotationAngleUnits=deg  RotationArbitraryAxis=[0 0 1]  RotationSequenceAxes=FollowerAxes  RotationSequence=XYX  RotationSequenceAngles=[0 0 0]  RotationSequenceAnglesUnits=deg  RotationMatrix=[1 0 0; 0 1 0; 0 0 1]  Quaternion=[1 0 0 0]  TranslationMethod=Cartesian  TranslationCartesianOffset=hp_in_r_ua.*rhs_hp  TranslationCartesianOffsetUnits=m  TranslationStandardAxis=+Z  TranslationStandardOffset=0  TranslationStandardOffsetUnits=m  TranslationROffset=0  TranslationROffsetUnits=m  TranslationThetaOffset=0  TranslationThetaOffsetUnits=deg  TranslationZOffset=0  TranslationZOffsetUnits=m
  Vis HP LAf : sm_lib/Body Elements/Spherical Solid  SphereRadius=size_hp  SphereRadiusUnits=m  ExportEntireGeometry=off  InertiaType=CalculateFromGeometry  BasedOnType=Density  Density=0  DensityUnits=kg/m^3  Mass=1  MassUnits=kg  CenterOfMass=[0 0 0]  CenterOfMassUnits=m  MomentsOfInertia=[1 1 1]  MomentsOfInertiaUnits=kg*m^2  ProductsOfInertia=[0 0 0]  ProductsOfInertiaUnits=kg*m^2  GraphicType=FromGeometry  MarkerShape=Sphere  MarkerSize=10  GraphicVisPropType=SimpleVisualProperties  GraphicDiffuseColor=clr_hp  GraphicOpacity=opc_hp  GraphicSpecularColor=[0.5 0.5 0.5 1.0]  GraphicAmbientColor=[0.15 0.15 0.15 1.0]  GraphicEmissiveColor=[0.0 0.0 0.0 1.0]  GraphicShininess=75  DoExposeReferenceFrame=on  SerializedFrames=<Frames/>
  Vis HP LAr : sm_lib/Body Elements/Spherical Solid  SphereRadius=size_hp  SphereRadiusUnits=m  ExportEntireGeometry=off  InertiaType=CalculateFromGeometry  BasedOnType=Density  Density=0  DensityUnits=kg/m^3  Mass=1  MassUnits=kg  CenterOfMass=[0 0 0]  CenterOfMassUnits=m  MomentsOfInertia=[1 1 1]  MomentsOfInertiaUnits=kg*m^2  ProductsOfInertia=[0 0 0]  ProductsOfInertiaUnits=kg*m^2  GraphicType=FromGeometry  MarkerShape=Sphere  MarkerSize=10  GraphicVisPropType=SimpleVisualProperties  GraphicDiffuseColor=clr_hp  GraphicOpacity=opc_hp  GraphicSpecularColor=[0.5 0.5 0.5 1.0]  GraphicAmbientColor=[0.15 0.15 0.15 1.0]  GraphicEmissiveColor=[0.0 0.0 0.0 1.0]  GraphicShininess=75  DoExposeReferenceFrame=on  SerializedFrames=<Frames/>
  Vis HP Shock : sm_lib/Body Elements/Spherical Solid  SphereRadius=size_hp  SphereRadiusUnits=m  ExportEntireGeometry=off  InertiaType=CalculateFromGeometry  BasedOnType=Density  Density=0  DensityUnits=kg/m^3  Mass=1  MassUnits=kg  CenterOfMass=[0 0 0]  CenterOfMassUnits=m  MomentsOfInertia=[1 1 1]  MomentsOfInertiaUnits=kg*m^2  ProductsOfInertia=[0 0 0]  ProductsOfInertiaUnits=kg*m^2  GraphicType=FromGeometry  MarkerShape=Sphere  MarkerSize=10  GraphicVisPropType=SimpleVisualProperties  GraphicDiffuseColor=clr_hp  GraphicOpacity=opc_hp  GraphicSpecularColor=[0.5 0.5 0.5 1.0]  GraphicAmbientColor=[0.15 0.15 0.15 1.0]  GraphicEmissiveColor=[0.0 0.0 0.0 1.0]  GraphicShininess=75  DoExposeReferenceFrame=on  SerializedFrames=<Frames/>
  Vis HP UAf : sm_lib/Body Elements/Spherical Solid  SphereRadius=size_hp  SphereRadiusUnits=m  ExportEntireGeometry=off  InertiaType=CalculateFromGeometry  BasedOnType=Density  Density=0  DensityUnits=kg/m^3  Mass=1  MassUnits=kg  CenterOfMass=[0 0 0]  CenterOfMassUnits=m  MomentsOfInertia=[1 1 1]  MomentsOfInertiaUnits=kg*m^2  ProductsOfInertia=[0 0 0]  ProductsOfInertiaUnits=kg*m^2  GraphicType=FromGeometry  MarkerShape=Sphere  MarkerSize=10  GraphicVisPropType=SimpleVisualProperties  GraphicDiffuseColor=clr_hp  GraphicOpacity=opc_hp  GraphicSpecularColor=[0.5 0.5 0.5 1.0]  GraphicAmbientColor=[0.15 0.15 0.15 1.0]  GraphicEmissiveColor=[0.0 0.0 0.0 1.0]  GraphicShininess=75  DoExposeReferenceFrame=on  SerializedFrames=<Frames/>
  Vis HP UAr : sm_lib/Body Elements/Spherical Solid  SphereRadius=size_hp  SphereRadiusUnits=m  ExportEntireGeometry=off  InertiaType=CalculateFromGeometry  BasedOnType=Density  Density=0  DensityUnits=kg/m^3  Mass=1  MassUnits=kg  CenterOfMass=[0 0 0]  CenterOfMassUnits=m  MomentsOfInertia=[1 1 1]  MomentsOfInertiaUnits=kg*m^2  ProductsOfInertia=[0 0 0]  ProductsOfInertiaUnits=kg*m^2  GraphicType=FromGeometry  MarkerShape=Sphere  MarkerSize=10  GraphicVisPropType=SimpleVisualProperties  GraphicDiffuseColor=clr_hp  GraphicOpacity=opc_hp  GraphicSpecularColor=[0.5 0.5 0.5 1.0]  GraphicAmbientColor=[0.15 0.15 0.15 1.0]  GraphicEmissiveColor=[0.0 0.0 0.0 1.0]  GraphicShininess=75  DoExposeReferenceFrame=on  SerializedFrames=<Frames/>
  UA : PMIOPort  Side=Left
  Shock : PMIOPort  Port=2  Side=Left
  LA : PMIOPort  Port=3  Side=Left
  Ref : PMIOPort  Port=4  Side=Right
  connections:
  Transform LAf/RConn1 -- Transform Align LAf LAr/LConn1
  Transform Align LAr LAf/LConn1 -- Transform LAr/RConn1
  Transform Align UAr UAf/RConn1 -- Vis HP UAr/RConn1 -- Simscape Bus UA/LConn3 -- Transform UAc/LConn1
  Transform Align UAr UAf/LConn1 -- Transform UAr/RConn1
  Transform UAf/RConn1 -- Transform Align UAf UAr/LConn1
  Vis HP Shock/RConn1 -- Shock/RConn1 -- Transform HP Shock/RConn1
  Simscape Bus UA/LConn1 -- Vis HP UAf/RConn1 -- Transform Align UAf UAr/RConn1
  Vis HP LAr/RConn1 -- Transform Align LAr LAf/RConn1 -- Transform LAc/LConn1 -- Simscape Bus LA/LConn3
  Vis HP LAf/RConn1 -- Transform Align LAf LAr/RConn1 -- Simscape Bus LA/LConn1
  Ref/RConn1 -- Transform UAf/LConn1 -- Transform UAr/LConn1 -- Transform HP Shock/LConn1 -- Transform LAf/LConn1 -- Transform LAr/LConn1
  Simscape Bus UA/LConn2 -- Transform UAc/RConn1
  UA/RConn1 -- Simscape Bus UA/RConn1
  Simscape Bus LA/LConn2 -- Transform LAc/RConn1
  Simscape Bus LA/RConn1 -- LA/RConn1

== system Linkage_DW_A/DoubleWishboneA/LA Upright ==
  No Steer : Subsystem  VariantControl=No_Steer
      mask Display: image('sm_car_variant_universal.png');
  Steer : Subsystem  VariantControl=Steer
      mask Display: image('sm_car_variant_spherical.png');
  F : PMIOPort  Side=Right
  " B" : PMIOPort  Port=2  Side=Left

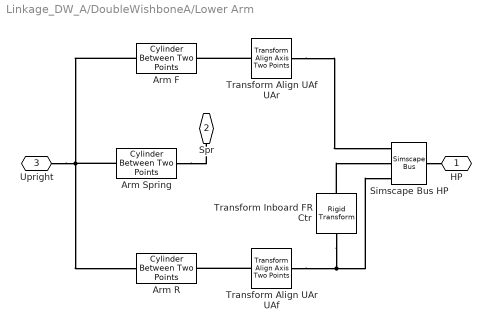
== system Linkage_DW_A/DoubleWishboneA/Lower Arm ==
  Arm F : Suspension_Utilities/Cylinder Between Two Points  hp_b=hp_in_f.*rhs_hp  hp_f=hp_out.*rhs_hp  Mass=la_mass/2  clr_solid=clr_la  opc_solid=opc_la  rad_solid=radius_la
      settings: SourceProductName=SmCar - Suspension Utilites
  Arm R : Suspension_Utilities/Cylinder Between Two Points  hp_b=hp_in_r.*rhs_hp  hp_f=hp_out.*rhs_hp  Mass=la_mass/2  clr_solid=clr_la  opc_solid=opc_la  rad_solid=radius_la
      settings: SourceProductName=SmCar - Suspension Utilites
  Arm Spring : Suspension_Utilities/Cylinder Between Two Points  hp_b=hp_spr.*rhs_hp  hp_f=hp_out.*rhs_hp  Mass=0  clr_solid=clr_la  opc_solid=opc_la  rad_solid=radius_la
      settings: SourceProductName=SmCar - Suspension Utilites
  Simscape Bus HP : SimscapeBus  HierarchyStrings=Af;Ac;Ar
  Transform Align UAf UAr : Suspension_Utilities/Transform Align Axis Two Points  hp_b=hp_in_r.*rhs_hp  hp_t=hp_in_f.*rhs_hp  popup_f_axis=+Z
      settings: SourceProductName=SmCar - Suspension Utilites
  Transform Align UAr UAf : Suspension_Utilities/Transform Align Axis Two Points  hp_b=hp_in_r.*rhs_hp  hp_t=hp_in_f.*rhs_hp  popup_f_axis=+Z
      settings: SourceProductName=SmCar - Suspension Utilites
  Transform Inboard FR Ctr : sm_lib/Frames and Transforms/Rigid Transform  RotationMethod=None  FollAlignAxisA=+X  BaseAlignAxisA=+Y  FollAlignAxisB=+Y  BaseAlignAxisB=+Z  RotationStandardAxis=+Z  RotationAngle=0.0  RotationAngleUnits=deg  RotationArbitraryAxis=[0 0 1]  RotationSequenceAxes=FollowerAxes  RotationSequence=XYX  RotationSequenceAngles=[0 0 0]  RotationSequenceAnglesUnits=deg  RotationMatrix=[1 0 0; 0 1 0; 0 0 1]  Quaternion=[1 0 0 0]  TranslationMethod=StandardAxis  TranslationCartesianOffset=[0 0 0]  TranslationCartesianOffsetUnits=m  TranslationStandardAxis=+Z  TranslationStandardOffset=norm(hp_in_f-hp_in_r)/2  TranslationStandardOffsetUnits=m  TranslationROffset=0  TranslationROffsetUnits=m  TranslationThetaOffset=0  TranslationThetaOffsetUnits=deg  TranslationZOffset=0  TranslationZOffsetUnits=m
  HP : PMIOPort  Side=Right
  Spr : PMIOPort  Port=2  Side=Left
  Upright : PMIOPort  Port=3  Side=Left
  connections:
  Transform Align UAf UAr/RConn1 -- Simscape Bus HP/LConn1
  Transform Align UAf UAr/LConn1 -- Arm F/LConn1
  Transform Align UAr UAf/LConn1 -- Arm R/LConn1
  Arm Spring/RConn1 -- Upright/RConn1 -- Arm R/RConn1 -- Arm F/RConn1
  Arm Spring/LConn1 -- Spr/RConn1
  Simscape Bus HP/RConn1 -- HP/RConn1
  Transform Inboard FR Ctr/RConn1 -- Simscape Bus HP/LConn2
  Transform Inboard FR Ctr/LConn1 -- Simscape Bus HP/LConn3 -- Transform Align UAr UAf/RConn1

== system Linkage_DW_A/DoubleWishboneA/Track Rod ==
  No Track Rod : Subsystem  VariantControl=No_Steer
      mask Display: disp(' ');
  Track Rod : Subsystem  VariantControl=Steer  mask{popup_leftRight=Left, hp_in=hp_in_rod, hp_out=hp_upr_rod, rod_mass=rod_mass, clr_conn_rod=clr_conn_rod, opc_conn_rod=opc_conn_rod, size_conn_rod=size_conn_rod, clr_rod=clr_rod, opc_rod=opc_rod, radius_rod=radius_rod}
      mask prompts: popup_leftRight "Left/Right"; hp_in "Inboard [xyz] (m)"; hp_out "Outboard [xyz] (m)"; rod_mass "Mass (kg)"
      mask init:
      | if(popup_leftRight == 1)
      |     rhs_rod = 1;
      | elseif(popup_leftRight == 2)
      |     rhs_rod = -1;
      | end
      | 
      | % Calculate lengths
      | %%%rod_len = norm(hp_out-hp_in);
      mask TypeOptions popup_leftRight: Left | Right
      mask TypeOptions rod_mass: Rod/Mass
      mask TypeOptions clr_conn_rod:
      | Vis
      | Upright
      | Steer/GraphicDiffuseColor | Vis
      | Rack
      | Rod/GraphicDiffuseColor
      mask TypeOptions opc_conn_rod:
      | Vis
      | Upright
      | Steer/GraphicOpacity | Vis
      | Rack
      | Rod/GraphicOpacity
      mask TypeOptions clr_rod: Rod/clr_solid
      mask TypeOptions opc_rod: Rod/opc_solid
      mask TypeOptions radius_rod: Rod/rad_solid
      mask DialogControl cont_rod Prompt: Rod
      mask DialogControl grp_rod Prompt: Rod
      mask DialogControl cont_vis_rod Prompt: Visualization
      mask DialogControl text_clr_rod Prompt: Color [RGB]
      mask DialogControl text_opc_rod Prompt: Opac. (0-1)
      mask DialogControl text_size_rod Prompt: Size (m)
      mask DialogControl text_conn_rod Prompt: Connections
      mask DialogControl text_rod_rod Prompt: Rod
      mask Display: image('sm_car_linkage_trackrod_IMAGE.png');
  " Steer" : PMIOPort  Side=Right
  " Upr" : PMIOPort  Port=2  Side=Left
